simulink model "PMSM_MC_2025a"  (R2025a)
settings: Solver=FixedStepDiscrete  StartTime=0.0  StopTime=10.0  FixedStep=0.00005  RelTol=1e-3
values from neighbouring files (symbols this model uses):
  MC_DCurrLopKi_CFG = 0.008293758    [PMSM_MC_Data_2025a.sldd]
  MC_DCurrLopKp_CFG = 0.0870848    [PMSM_MC_Data_2025a.sldd]
  MC_MotModeDebug_CFG = 255.0    [PMSM_MC_Data_2025a.sldd]
  MC_POLE_NUM_CFG = 7.0    [PMSM_MC_Data_2025a.sldd]
  MC_QCurrLopKi_CFG = 0.008293758    [PMSM_MC_Data_2025a.sldd]
  MC_QCurrLopKp_CFG = 0.0870848    [PMSM_MC_Data_2025a.sldd]
  MC_SpdLopKi_CFG = 1.0E-5    [PMSM_MC_Data_2025a.sldd]
  MC_SpdLopKp_CFG = 0.002    [PMSM_MC_Data_2025a.sldd]
libraries: simulink x10, slpidlib x3
settings Model: DataDictionary=PMSM_MC_Data_2025a.sldd  Creator=EDY  LastModifiedBy=xiaoy
settings OptimizationCC: DefaultParameterBehavior=Inlined  EnhancedBackFolding=on  PassReuseOutputArgsAs=Individual arguments  ZeroExternalMemoryAtStartup=off  ZeroInternalMemoryAtStartup=off  OptimizeBlockOrder=speed  DifferentSizesBufferReuse=on  OptimizationCustomize=off  EfficientTunableParamExpr=on
settings DebuggingCC: ParameterTunabilityLossMsg=error
settings SFSimCC: MATLABDynamicMemAlloc=off
settings RTWCC: SystemTargetFile=ert.tlc  GenCodeOnly=on  TemplateMakefile=ert_default_tmf  GenerateReport=on  LaunchReport=on  Description=Embedded Coder
settings CodeAppCC: ForceParamTrailComments=on  IgnoreCustomStorageClasses=off  OperatorAnnotations=on  SimulinkDataObjDesc=on  SFDataObjDesc=on  InsertBlockDesc=on
settings ERTTargetCC: ExtModeTransport=0.0  ExtModeStaticAlloc=off  ExtModeMexFile=ext_comm  ExtModeIntrfLevel=Level1  ERTCustomFileTemplate=example_file_process.tlc  DynamicArrayContainerType=coder::array  TargetLangStandard=C99 (ISO)  GenerateSampleERTMain=on

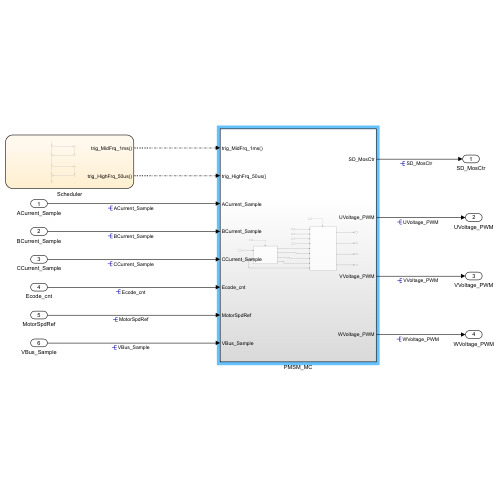
[thumbnail: Simulink's stored preview of the top-level diagram]
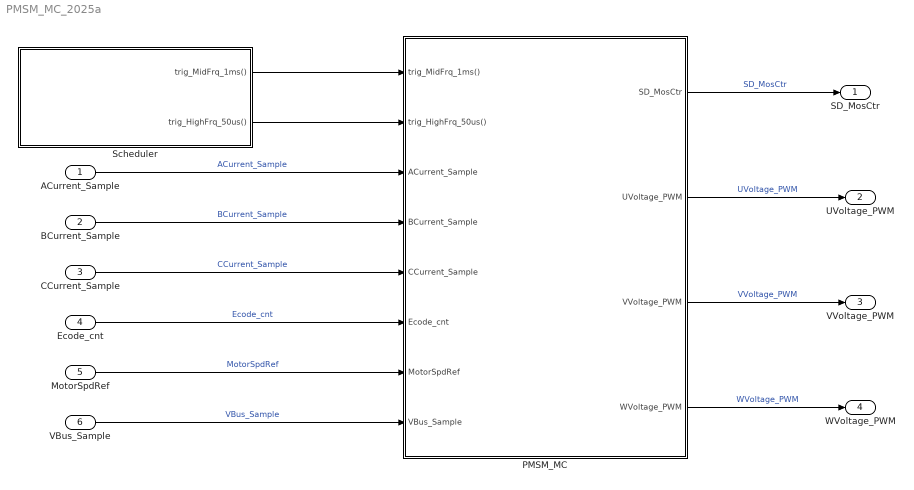
== system PMSM_MC_2025a ==
  ACurrent_Sample : Inport
  BCurrent_Sample : Inport  Port=2
  CCurrent_Sample : Inport  Port=3
  Ecode_cnt : Inport  Port=4
  MotorSpdRef : Inport  Port=5
  VBus_Sample : Inport  Port=6
  PMSM_MC : Subsystem
  Scheduler : Stateflow chart  TreatAsAtomicUnit=on
  SD_MosCtr : Outport
  UVoltage_PWM : Outport  Port=2
  VVoltage_PWM : Outport  Port=3
  WVoltage_PWM : Outport  Port=4
  wires:
  Scheduler/1(trig_MidFrq_1ms()) -> PMSM_MC/1(trig_MidFrq_1ms())
  Scheduler/2(trig_HighFrq_50us()) -> PMSM_MC/2(trig_HighFrq_50us())
  VBus_Sample/1 -> PMSM_MC/8(VBus_Sample)  "VBus_Sample"
  MotorSpdRef/1 -> PMSM_MC/7(MotorSpdRef)  "MotorSpdRef"
  Ecode_cnt/1 -> PMSM_MC/6(Ecode_cnt)  "Ecode_cnt"
  CCurrent_Sample/1 -> PMSM_MC/5(CCurrent_Sample)  "CCurrent_Sample"
  BCurrent_Sample/1 -> PMSM_MC/4(BCurrent_Sample)  "BCurrent_Sample"
  ACurrent_Sample/1 -> PMSM_MC/3(ACurrent_Sample)  "ACurrent_Sample"
  PMSM_MC/2(UVoltage_PWM) -> UVoltage_PWM/1  "UVoltage_PWM"
  PMSM_MC/1(SD_MosCtr) -> SD_MosCtr/1  "SD_MosCtr"
  PMSM_MC/3(VVoltage_PWM) -> VVoltage_PWM/1  "VVoltage_PWM"
  PMSM_MC/4(WVoltage_PWM) -> WVoltage_PWM/1  "WVoltage_PWM"

== system PMSM_MC_2025a/PMSM_MC ==
  trig_MidFrq_1ms() : Inport
  trig_HighFrq_50us() : Inport  Port=2
  ACurrent_Sample : Inport  Port=3
  BCurrent_Sample : Inport  Port=4
  CCurrent_Sample : Inport  Port=5
  Ecode_cnt : Inport  Port=6
  MotorSpdRef : Inport  Port=7
  VBus_Sample : Inport  Port=8
  MC_HighFrqTask : Subsystem  TreatAsAtomicUnit=on
  MC_LowFrqTask : Subsystem  TreatAsAtomicUnit=on
  SD_MosCtr : Outport
  UVoltage_PWM : Outport  Port=2
  VVoltage_PWM : Outport  Port=3
  WVoltage_PWM : Outport  Port=4
  wires:
  trig_MidFrq_1ms()/1 -> MC_LowFrqTask/Trigger
  trig_HighFrq_50us()/1 -> MC_HighFrqTask/Trigger
  Ecode_cnt/1 -> MC_HighFrqTask/9(Ecode_cnt), MC_LowFrqTask/2(Ecode_cnt)
  MotorSpdRef/1 -> MC_LowFrqTask/1(MotorSpdRef)
  ACurrent_Sample/1 -> MC_HighFrqTask/1(ACurrent_Sample)
  BCurrent_Sample/1 -> MC_HighFrqTask/2(BCurrent_Sample)
  CCurrent_Sample/1 -> MC_HighFrqTask/3(CCurrent_Sample)
  VBus_Sample/1 -> MC_HighFrqTask/4(VBus_Sample)
  MC_LowFrqTask/1(QAxiCurrent_Ref) -> MC_HighFrqTask/5(QAxiCurrent_Ref)
  MC_LowFrqTask/2(MotCalThetae) -> MC_HighFrqTask/6(MotCalThetae)
  MC_LowFrqTask/3(MotOffset) -> MC_HighFrqTask/7(MotOffset)
  MC_LowFrqTask/4(MotCtrMode) -> MC_HighFrqTask/8(MotCtrMode)
  MC_HighFrqTask/1(SD_MosCtr) -> SD_MosCtr/1
  MC_HighFrqTask/2(UVoltage_PWM) -> UVoltage_PWM/1
  MC_HighFrqTask/3(VVoltage_PWM) -> VVoltage_PWM/1
  MC_HighFrqTask/4(WVoltage_PWM) -> WVoltage_PWM/1

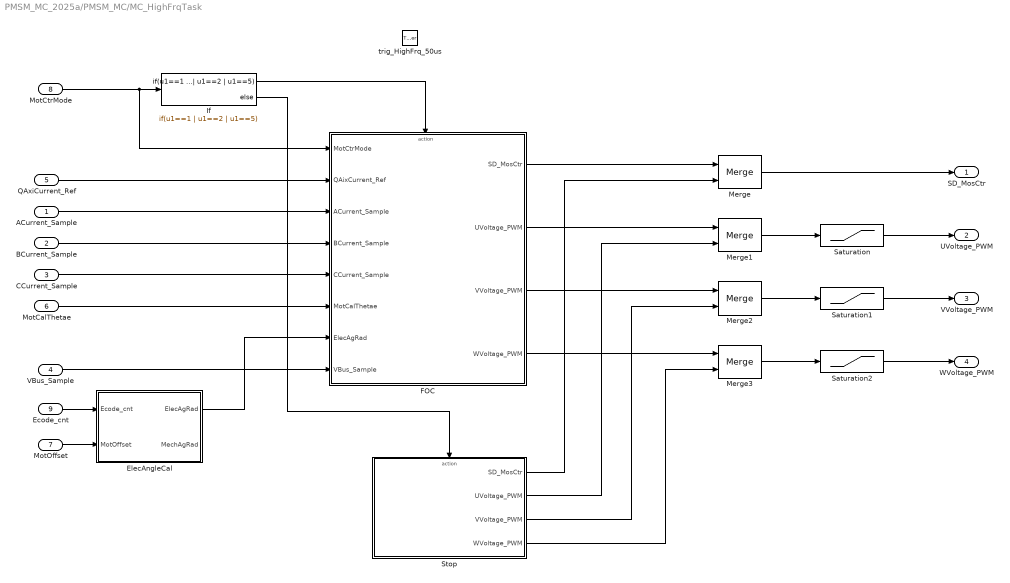
== system PMSM_MC_2025a/PMSM_MC/MC_HighFrqTask ==
  ACurrent_Sample : Inport
  BCurrent_Sample : Inport  Port=2
  CCurrent_Sample : Inport  Port=3
  VBus_Sample : Inport  Port=4
  QAxiCurrent_Ref : Inport  Port=5
  MotCalThetae : Inport  Port=6
  MotOffset : Inport  Port=7
  MotCtrMode : Inport  Port=8
  Ecode_cnt : Inport  Port=9
  trig_HighFrq_50us : TriggerPort  TriggerType=function-call  VariantControl=(inherit)
  ElecAngleCal : Subsystem
  FOC : Subsystem
  If : If  IfExpression=u1==1 | u1==2 | u1==5
  Merge{,1..3} (4 alike) : Merge
  Saturation : Saturate  UpperLimit=0.95  LowerLimit=0
      settings: AttributesFormatString=|
      | Upper = %<UpperLimit>
      | Lower = %<LowerLimit>
  Saturation1 : Saturate  UpperLimit=0.95  LowerLimit=0
      settings: AttributesFormatString=|
      | Upper = %<UpperLimit>
      | Lower = %<LowerLimit>
  Saturation2 : Saturate  UpperLimit=0.95  LowerLimit=0
      settings: AttributesFormatString=|
      | Upper = %<UpperLimit>
      | Lower = %<LowerLimit>
  Stop : Subsystem  TreatAsAtomicUnit=on
  SD_MosCtr : Outport
  UVoltage_PWM : Outport  Port=2
  VVoltage_PWM : Outport  Port=3
  WVoltage_PWM : Outport  Port=4
  wires:
  MotCtrMode/1 -> FOC/1(MotCtrMode), If/1
  If/1 -> FOC/Action
  If/2 -> Stop/Action
  FOC/1(SD_MosCtr) -> Merge/1
  FOC/2(UVoltage_PWM) -> Merge1/1
  FOC/3(VVoltage_PWM) -> Merge2/1
  FOC/4(WVoltage_PWM) -> Merge3/1
  Merge/1 -> SD_MosCtr/1
  Stop/1(SD_MosCtr) -> Merge/2
  Stop/2(UVoltage_PWM) -> Merge1/2
  Stop/3(VVoltage_PWM) -> Merge2/2
  Stop/4(WVoltage_PWM) -> Merge3/2
  Merge1/1 -> Saturation/1
  Merge3/1 -> Saturation2/1
  Merge2/1 -> Saturation1/1
  Saturation/1 -> UVoltage_PWM/1
  Saturation1/1 -> VVoltage_PWM/1
  Saturation2/1 -> WVoltage_PWM/1
  MotOffset/1 -> ElecAngleCal/2(MotOffset)
  Ecode_cnt/1 -> ElecAngleCal/1(Ecode_cnt)
  ACurrent_Sample/1 -> FOC/3(ACurrent_Sample)
  BCurrent_Sample/1 -> FOC/4(BCurrent_Sample)
  CCurrent_Sample/1 -> FOC/5(CCurrent_Sample)
  QAxiCurrent_Ref/1 -> FOC/2(QAixCurrent_Ref)
  MotCalThetae/1 -> FOC/6(MotCalThetae)
  VBus_Sample/1 -> FOC/8(VBus_Sample)
  ElecAngleCal/1(ElecAgRad) -> FOC/7(ElecAgRad)

== system PMSM_MC_2025a/PMSM_MC/MC_LowFrqTask ==
  MotorSpdRef : Inport
  Ecode_cnt : Inport  Port=2
  trig_MidFrq_1ms : TriggerPort  TriggerType=function-call  VariantControl=(inherit)
  MotModeCtr : Subsystem
  MotSpdCal : Subsystem
  SpdLoop : Subsystem
  QAxiCurrent_Ref : Outport
  MotCalThetae : Outport  Port=2
  MotOffset : Outport  Port=3
  MotCtrMode : Outport  Port=4
  wires:
  SpdLoop/1(QAxiCurrent_Ref) -> QAxiCurrent_Ref/1
  MotorSpdRef/1 -> SpdLoop/2(MotorSpdRef), MotModeCtr/2(MotorSpdRef)
  Ecode_cnt/1 -> MotSpdCal/1(Ecode_cnt), MotModeCtr/1(Ecode_cnt)
  MotSpdCal/1(MotorActSpd) -> SpdLoop/3(MotorActSpd)  "MotorActSpd"
  MotModeCtr/3(MotCtrMode) -> SpdLoop/1(MotCtrMode), MotCtrMode/1
  MotModeCtr/2(MotCalThetae) -> MotCalThetae/1
  MotModeCtr/1(MotOffset) -> MotOffset/1

== system PMSM_MC_2025a/PMSM_MC/MC_HighFrqTask/ElecAngleCal ==
  Ecode_cnt : Inport
  MotOffset : Inport  Port=2
  Add : Sum  Inputs=+-
  AngleCal : Subsystem
  Demux : Demux  Outputs=2
  ElecAgRad : Outport
  MechAgRad : Outport  Port=2
  wires:
  Ecode_cnt/1 -> Add/1
  MotOffset/1 -> Add/2
  Add/1 -> AngleCal/1(Ecode_CntCorrect)
  AngleCal/1(Theta) -> Demux/1
  Demux/1 -> MechAgRad/1
  Demux/2 -> ElecAgRad/1

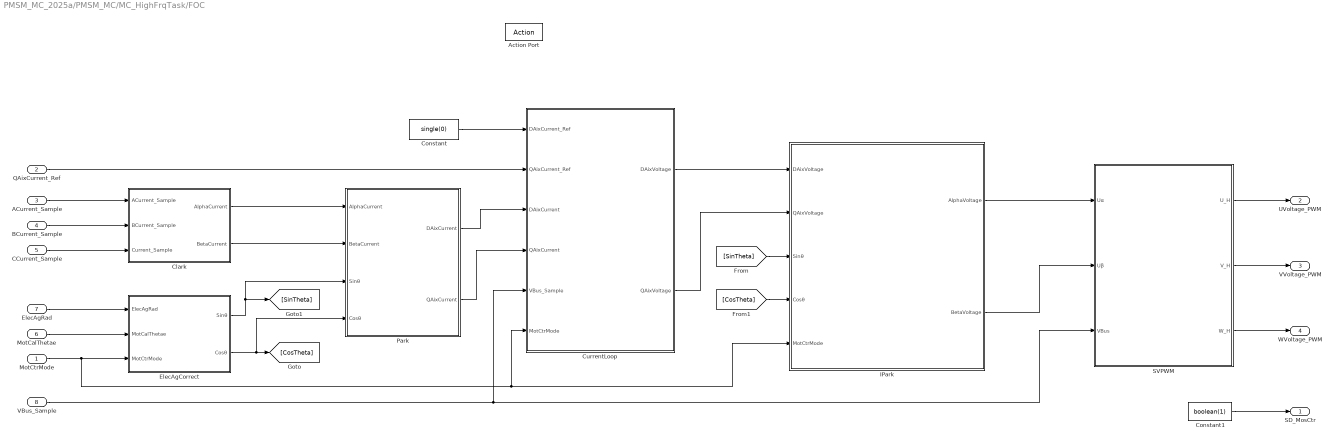
== system PMSM_MC_2025a/PMSM_MC/MC_HighFrqTask/FOC ==
  MotCtrMode : Inport
  QAixCurrent_Ref : Inport  Port=2
  ACurrent_Sample : Inport  Port=3
  BCurrent_Sample : Inport  Port=4
  CCurrent_Sample : Inport  Port=5
  MotCalThetae : Inport  Port=6
  ElecAgRad : Inport  Port=7
  VBus_Sample : Inport  Port=8
  Action Port : ActionPort  ActionPortLabel=if(u1==1 | u1==2 | u1==5)
  Clark : Subsystem
  Constant : Constant  Value=single(0)
  Constant1 : Constant  Value=boolean(1)
  CurrentLoop : Subsystem
  ElecAgCorrect : Subsystem
  IPark : Subsystem
  Park : Subsystem
  SVPWM : Subsystem
  SD_MosCtr : Outport
  UVoltage_PWM : Outport  Port=2
  VVoltage_PWM : Outport  Port=3
  WVoltage_PWM : Outport  Port=4
  wires:
  Clark/2(BetaCurrent) -> Park/2(BetaCurrent)
  Clark/1(AlphaCurrent) -> Park/1(AlphaCurrent)
  Park/1(DAixCurrent) -> CurrentLoop/3(DAixCurrent)
  QAixCurrent_Ref/1 -> CurrentLoop/2(QAixCurrent_Ref)
  Constant/1 -> CurrentLoop/1(DAixCurrent_Ref)
  CurrentLoop/1(DAixVoltage) -> IPark/1(DAixVoltage)
  CurrentLoop/2(QAixVoltage) -> IPark/2(QAixVoltage)
  Park/2(QAixCurrent) -> CurrentLoop/4(QAixCurrent)
  ACurrent_Sample/1 -> Clark/1(ACurrent_Sample)
  BCurrent_Sample/1 -> Clark/2(BCurrent_Sample)
  CCurrent_Sample/1 -> Clark/3(Current_Sample)
  ElecAgRad/1 -> ElecAgCorrect/1(ElecAgRad)
  MotCalThetae/1 -> ElecAgCorrect/2(MotCalThetae)
  MotCtrMode/1 -> CurrentLoop/6(MotCtrMode), IPark/5(MotCtrMode), ElecAgCorrect/3(MotCtrMode)
  ElecAgCorrect/1(Sinθ) -> Park/3(Sinθ), [SinTheta]
  ElecAgCorrect/2(Cosθ) -> [CosTheta], Park/4(Cosθ)
  [SinTheta] -> IPark/3(Sinθ)
  [CosTheta] -> IPark/4(Cosθ)
  VBus_Sample/1 -> CurrentLoop/5(VBus_Sample), SVPWM/3(VBus)
  IPark/1(AlphaVoltage) -> SVPWM/1(Uα)
  IPark/2(BetaVoltage) -> SVPWM/2(Uβ)
  SVPWM/1(U_H) -> UVoltage_PWM/1
  SVPWM/2(V_H) -> VVoltage_PWM/1
  SVPWM/3(W_H) -> WVoltage_PWM/1
  Constant1/1 -> SD_MosCtr/1

== system PMSM_MC_2025a/PMSM_MC/MC_HighFrqTask/Stop ==
  Action Port : ActionPort  ActionPortLabel=else
  Constant : Constant  Value=single(0)
  Constant1 : Constant  Value=boolean(0)
  SD_MosCtr : Outport
  UVoltage_PWM : Outport  Port=2
  VVoltage_PWM : Outport  Port=3
  WVoltage_PWM : Outport  Port=4
  wires:
  Constant/1 -> WVoltage_PWM/1, VVoltage_PWM/1, UVoltage_PWM/1
  Constant1/1 -> SD_MosCtr/1

== system PMSM_MC_2025a/PMSM_MC/MC_LowFrqTask/MotModeCtr ==
  Ecode_cnt : Inport
  MotorSpdRef : Inport  Port=2
  Chart : Stateflow chart  TreatAsAtomicUnit=on
  Compare To Constant : simulink/Logic and Bit Operations/Compare To Constant  relop=~=  const=255  OutDataTypeStr=boolean
  Constant : Constant  Value=MC_MotModeDebug_CFG
  Switch : Switch  Criteria=u2 ~= 0  SaturateOnIntegerOverflow=off  InputSameDT=off
  MotOffset : Outport
  MotCalThetae : Outport  Port=2
  MotCtrMode : Outport  Port=3
  wires:
  Chart/2(MotOffset) -> MotOffset/1
  Chart/3(MotCalThetae) -> MotCalThetae/1
  Ecode_cnt/1 -> Chart/1(Ecode_cnt)
  MotorSpdRef/1 -> Chart/2(MotorSpdRef)
  Chart/1(MotCtrMode) -> Switch/3
  Switch/1 -> MotCtrMode/1
  Constant/1 -> Switch/1, Compare To Constant/1
  Compare To Constant/1 -> Switch/2

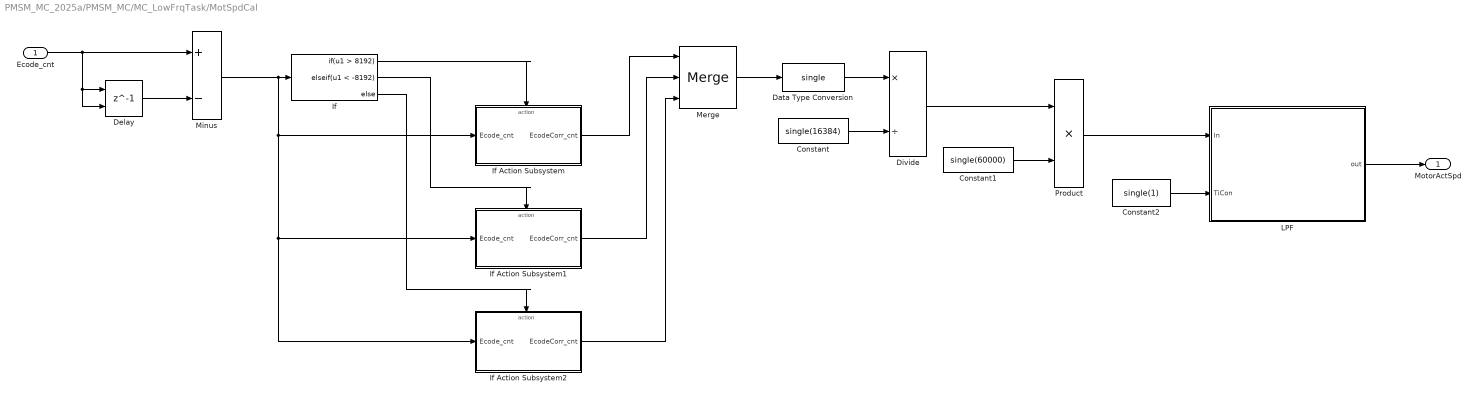
== system PMSM_MC_2025a/PMSM_MC/MC_LowFrqTask/MotSpdCal ==
  Ecode_cnt : Inport
  Constant : Constant  Value=single(16384)
  Constant1 : Constant  Value=single(60000)
  Constant2 : Constant  Value=single(1)
  Data Type Conversion : DataTypeConversion  OutDataTypeStr=single  SaturateOnIntegerOverflow=off  RndMeth=Floor
  Delay : Delay  DelayLength=1  InitialConditionSource=Input port
      settings: InputPortMap=u0,p4
  Divide : Product  Inputs=*/
  If : If  IfExpression=u1 > 8192  ElseIfExpressions=u1 < -8192
  If Action Subsystem : Subsystem  TreatAsAtomicUnit=on
  If Action Subsystem1 : Subsystem  TreatAsAtomicUnit=on
  If Action Subsystem2 : Subsystem  TreatAsAtomicUnit=on
  LPF : Subsystem
  Merge : Merge  Inputs=3
  Minus : Sum  Inputs=+-
  Product : Product
  MotorActSpd : Outport
  wires:
  Ecode_cnt/1 -> Delay/2, Delay/1, Minus/1
  Delay/1 -> Minus/2
  Data Type Conversion/1 -> Divide/1
  Constant/1 -> Divide/2
  Divide/1 -> Product/1
  Constant1/1 -> Product/2
  Product/1 -> LPF/1(In)
  Constant2/1 -> LPF/2(TiCon)
  LPF/1(out) -> MotorActSpd/1
  Minus/1 -> If Action Subsystem/1(Ecode_cnt), If Action Subsystem2/1(Ecode_cnt), If Action Subsystem1/1(Ecode_cnt), If/1
  If/1 -> If Action Subsystem/Action
  If/2 -> If Action Subsystem1/Action
  If/3 -> If Action Subsystem2/Action
  If Action Subsystem/1(EcodeCorr_cnt) -> Merge/1
  If Action Subsystem1/1(EcodeCorr_cnt) -> Merge/2
  If Action Subsystem2/1(EcodeCorr_cnt) -> Merge/3
  Merge/1 -> Data Type Conversion/1

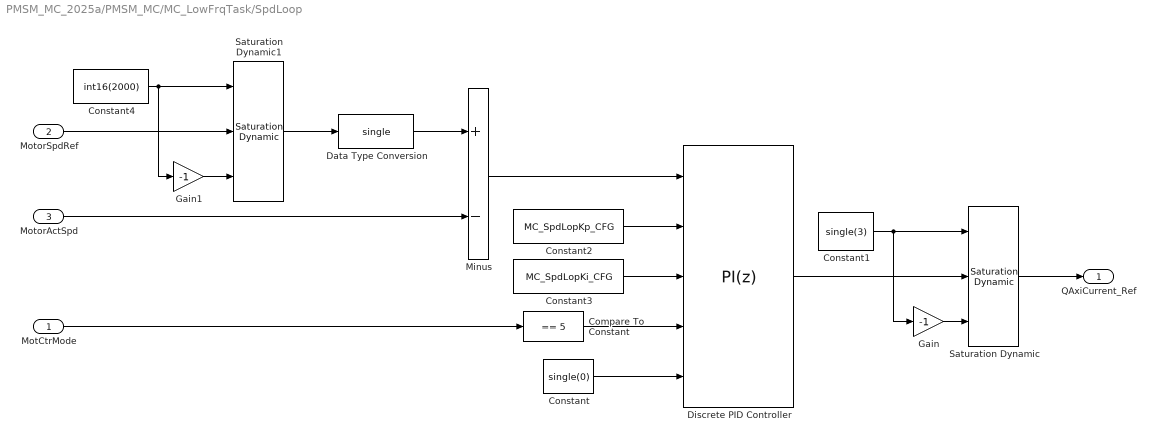
== system PMSM_MC_2025a/PMSM_MC/MC_LowFrqTask/SpdLoop ==
  MotCtrMode : Inport
  MotorSpdRef : Inport  Port=2
  MotorActSpd : Inport  Port=3
  Compare To Constant : simulink/Logic and Bit Operations/Compare To Constant  relop===  const=5  OutDataTypeStr=boolean
  Constant : Constant  Value=single(0)  OutDataTypeStr=single
  Constant1 : Constant  Value=single(3)
  Constant2 : Constant  Value=MC_SpdLopKp_CFG
  Constant3 : Constant  Value=MC_SpdLopKi_CFG
  Constant4 : Constant  Value=int16(2000)
  Data Type Conversion : DataTypeConversion  OutDataTypeStr=single  SaturateOnIntegerOverflow=off  RndMeth=Floor
  Discrete PID Controller : slpidlib/PID Controller  Controller=PI  Form=Parallel  TimeDomain=Discrete-time  UseExternalTs=off  SampleTime=-1  IntegratorMethod=Forward Euler  FilterMethod=Forward Euler  ControllerParametersSource=external  P=1  I=1  UseKiTs=on  D=0  UseExternalDerivativeSource=off  N=100  UseFilter=on  TunerSelectOption=Transfer Function Based (PID Tuner App)  InitialConditionSource=external  InitialConditionForIntegrator=0  InitialConditionForFilter=0  DifferentiatorICPrevScaledInput=0  ExternalReset=rising  TrackingMode=off  Kt=1  LimitOutput=off  SatLimitsSource=external  UpperSaturationLimit=inf  LowerSaturationLimit=-inf  LinearizeAsGain=off  AntiWindupMode=none  Kb=1  LimitIntegrator=on  UpperIntegratorSaturationLimit=3  LowerIntegratorSaturationLimit=-3  POutMin=[]  POutMax=[]  IOutMin=[]  IOutMax=[]  DOutMin=[]  DOutMax=[]  NOutMin=[]  NOutMax=[]  SumOutMin=[]  SumOutMax=[]  SaturationOutMin=[]  SaturationOutMax=[]  PParamMin=[]  PParamMax=[]  IParamMin=[]  IParamMax=[]  DParamMin=[]  DParamMax=[]  NParamMin=[]  NParamMax=[]  KbParamMin=[]  KbParamMax=[]  KtParamMin=[]  KtParamMax=[]  KbOutMin=[]  KbOutMax=[]  KtOutMin=[]  KtOutMax=[]  IntegratorOutMin=[]  IntegratorOutMax=[]  FilterOutMin=[]  FilterOutMax=[]  SumI1OutMin=[]  SumI1OutMax=[]  SumI2OutMin=[]  SumI2OutMax=[]  SumI3OutMin=[]  SumI3OutMax=[]  SumI4OutMin=[]  SumI4OutMax=[]  SumDOutMin=[]  SumDOutMax=[]  DifferentiatorOutMin=[]  DifferentiatorOutMax=[]  FilterDiffOutCoefMin=[]  FilterDiffOutCoefMax=[]  ReciprocalOutMin=[]  ReciprocalOutMax=[]  SumDenOutMin=[]  SumDenOutMax=[]  SumNumOutMin=[]  SumNumOutMax=[]  DivideOutMin=[]  DivideOutMax=[]  UdiffTsProdOutMin=[]  UdiffTsProdOutMax=[]  NTsProdOutMin=[]  NTsProdOutMax=[]  UintegralTsProdOutMin=[]  UintegralTsProdOutMax=[]  UngainTsProdOutMin=[]  UngainTsProdOutMax=[]  ClampingZeroOutDataTypeStr=Inherit: Inherit via back propagation  ClampingZeroOutMin=[]  ClampingZeroOutMax=[]  FilterDenConstantOutDataTypeStr=Inherit: Inherit via back propagation  FilterDenConstantOutMin=[]  FilterDenConstantOutMax=[]  PCopyOutDataTypeStr=Inherit: Inherit via back propagation  PCopyOutMin=[]  PCopyOutMax=[]  NCopyOutDataTypeStr=Inherit: Inherit via back propagation  NCopyOutMin=[]  NCopyOutMax=[]  IntegratorContinuousStateAttributes=''  IntegratorStateMustResolveToSignalObject=off  IntegratorRTWStateStorageClass=Auto  FilterContinuousStateAttributes=''  FilterStateMustResolveToSignalObject=off  FilterRTWStateStorageClass=Auto  ParallelPVariant=ExternalParameters  IdealPVariant=Disabled  IVariant=ExternalParameters  DVariant=Disabled  IntegratorVariant=Discrete  SatVariant=Disabled  AWVariant=Passthrough  PCopyVariant=Disabled  TRVariant=Disabled  FdbkBlocksVariant=Forward  IdealPFdbkVariant=Disabled  SatFdbkVariant=Disabled  DerivativeFilterVariant=Disabled  NVariant=Disabled  NCopyVariant=Disabled_SignalSpec  FilterICVariant=Disabled  IntegratorICVariant=ExternalICs  ExternalResetVariant=ExternalReset  TRSumVariant=Passthrough  SumFdbkVariant=Disabled  SumVariant=Sum_PI  TsampFilterVariant=InternalTs  TsampNgainVariant=Passthrough  TsampIntegralVariant=Disabled_SignalSpec  ExternalSaturationOutDataTypeStr=Inherit: Same as second input  DerivativeSourceVariant=Disabled  PreIntVariant=InternalPreInt
      settings: LibrarySourceBlock=simulink/Discrete/Discrete PID Controller
  Gain : Gain  Gain=-1
  Gain1 : Gain  Gain=-1
  Minus : Sum  Inputs=+-
  Saturation Dynamic : simulink/Discontinuities/Saturation Dynamic  OutMin=[]  OutMax=[]  OutDataTypeStr=Inherit: Same as second input  OutDataType=fixdt(1, 16)  OutScaling=2^-10  DoSatur=off
  Saturation Dynamic1 : simulink/Discontinuities/Saturation Dynamic  OutMin=[]  OutMax=[]  OutDataTypeStr=Inherit: Same as second input  OutDataType=fixdt(1, 16)  OutScaling=2^-10  DoSatur=off
  QAxiCurrent_Ref : Outport
  wires:
  Data Type Conversion/1 -> Minus/1
  Constant/1 -> Discrete PID Controller/5
  Discrete PID Controller/1 -> Saturation Dynamic/2
  Saturation Dynamic/1 -> QAxiCurrent_Ref/1
  Constant1/1 -> Saturation Dynamic/1, Gain/1
  Gain/1 -> Saturation Dynamic/3
  Minus/1 -> Discrete PID Controller/1
  Constant2/1 -> Discrete PID Controller/2
  Constant3/1 -> Discrete PID Controller/3
  MotorSpdRef/1 -> Saturation Dynamic1/2
  Saturation Dynamic1/1 -> Data Type Conversion/1
  Constant4/1 -> Gain1/1, Saturation Dynamic1/1
  Gain1/1 -> Saturation Dynamic1/3
  MotorActSpd/1 -> Minus/2
  Compare To Constant/1 -> Discrete PID Controller/4
  MotCtrMode/1 -> Compare To Constant/1

== system PMSM_MC_2025a/PMSM_MC/MC_HighFrqTask/ElecAngleCal/AngleCal ==
  Ecode_CntCorrect : Inport
  If : If  IfExpression=u1 == 1  ElseIfExpressions=u1 == -1
  If Action Subsystem : Subsystem  TreatAsAtomicUnit=on
  If Action Subsystem1 : Subsystem  TreatAsAtomicUnit=on
  If Action Subsystem2 : Subsystem  TreatAsAtomicUnit=on
  Merge : Merge  Inputs=3
  Sign : Signum
  Theta : Outport
  wires:
  Ecode_CntCorrect/1 -> If Action Subsystem1/1(Ecode_PhyVal), If Action Subsystem/1(Ecode_PhyVal), Sign/1
  Sign/1 -> If/1
  If/1 -> If Action Subsystem/Action
  If/2 -> If Action Subsystem1/Action
  If/3 -> If Action Subsystem2/Action
  If Action Subsystem1/1(Out1) -> Merge/2
  If Action Subsystem/1(Out1) -> Merge/1
  Merge/1 -> Theta/1
  If Action Subsystem2/1(Out1) -> Merge/3

== system PMSM_MC_2025a/PMSM_MC/MC_HighFrqTask/FOC/Clark ==
  ACurrent_Sample : Inport
  BCurrent_Sample : Inport  Port=2
  Current_Sample : Inport  Port=3
  Gain : Gain  Gain=0.57735
  Gain1 : Gain  Gain=0.57735
  Minus : Sum  Inputs=+-
  AlphaCurrent : Outport
  BetaCurrent : Outport  Port=2
  wires:
  ACurrent_Sample/1 -> AlphaCurrent/1
  Minus/1 -> BetaCurrent/1
  Gain1/1 -> Minus/2
  Gain/1 -> Minus/1
  BCurrent_Sample/1 -> Gain/1
  Current_Sample/1 -> Gain1/1

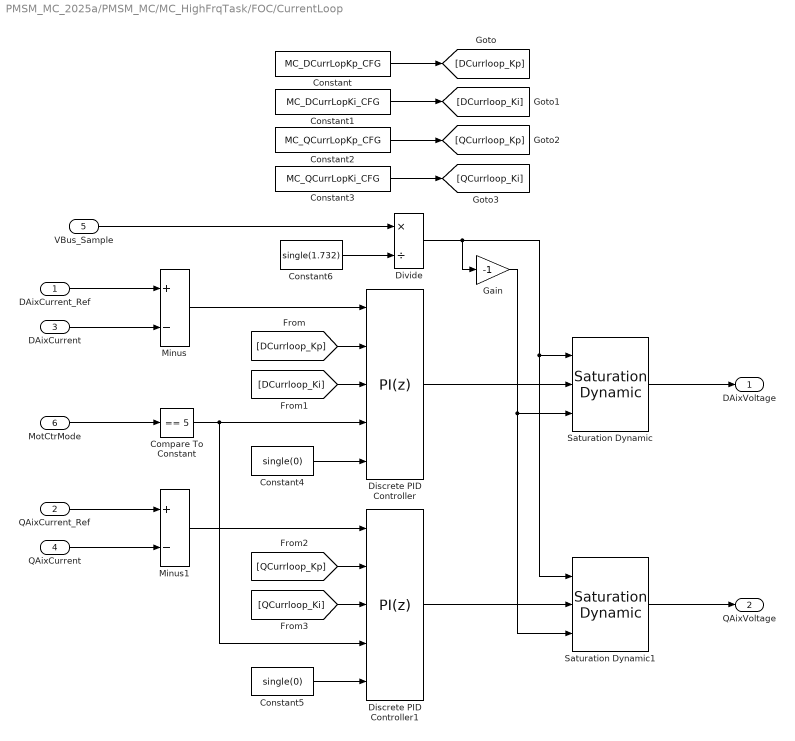
== system PMSM_MC_2025a/PMSM_MC/MC_HighFrqTask/FOC/CurrentLoop ==
  DAixCurrent_Ref : Inport
  QAixCurrent_Ref : Inport  Port=2
  DAixCurrent : Inport  Port=3
  QAixCurrent : Inport  Port=4
  VBus_Sample : Inport  Port=5
  MotCtrMode : Inport  Port=6
  Compare To Constant : simulink/Logic and Bit Operations/Compare To Constant  relop===  const=5  OutDataTypeStr=boolean
  Constant : Constant  Value=MC_DCurrLopKp_CFG
  Constant1 : Constant  Value=MC_DCurrLopKi_CFG
  Constant2 : Constant  Value=MC_QCurrLopKp_CFG
  Constant3 : Constant  Value=MC_QCurrLopKi_CFG
  Constant4 : Constant  Value=single(0)
  Constant5 : Constant  Value=single(0)
  Constant6 : Constant  Value=single(1.732)
  Discrete PID Controller : slpidlib/PID Controller  Controller=PI  Form=Parallel  TimeDomain=Discrete-time  UseExternalTs=off  SampleTime=-1  IntegratorMethod=Forward Euler  FilterMethod=Forward Euler  ControllerParametersSource=external  P=1  I=1  UseKiTs=on  D=0  UseExternalDerivativeSource=off  N=100  UseFilter=on  TunerSelectOption=Transfer Function Based (PID Tuner App)  InitialConditionSource=external  InitialConditionForIntegrator=0  InitialConditionForFilter=0  DifferentiatorICPrevScaledInput=0  ExternalReset=rising  TrackingMode=off  Kt=1  LimitOutput=off  SatLimitsSource=internal  UpperSaturationLimit=inf  LowerSaturationLimit=-inf  LinearizeAsGain=off  AntiWindupMode=none  Kb=1  LimitIntegrator=on  UpperIntegratorSaturationLimit=13  LowerIntegratorSaturationLimit=-13  POutMin=[]  POutMax=[]  IOutMin=[]  IOutMax=[]  DOutMin=[]  DOutMax=[]  NOutMin=[]  NOutMax=[]  SumOutMin=[]  SumOutMax=[]  SaturationOutMin=[]  SaturationOutMax=[]  PParamMin=[]  PParamMax=[]  IParamMin=[]  IParamMax=[]  DParamMin=[]  DParamMax=[]  NParamMin=[]  NParamMax=[]  KbParamMin=[]  KbParamMax=[]  KtParamMin=[]  KtParamMax=[]  KbOutMin=[]  KbOutMax=[]  KtOutMin=[]  KtOutMax=[]  IntegratorOutMin=[]  IntegratorOutMax=[]  FilterOutMin=[]  FilterOutMax=[]  SumI1OutMin=[]  SumI1OutMax=[]  SumI2OutMin=[]  SumI2OutMax=[]  SumI3OutMin=[]  SumI3OutMax=[]  SumI4OutMin=[]  SumI4OutMax=[]  SumDOutMin=[]  SumDOutMax=[]  DifferentiatorOutMin=[]  DifferentiatorOutMax=[]  FilterDiffOutCoefMin=[]  FilterDiffOutCoefMax=[]  ReciprocalOutMin=[]  ReciprocalOutMax=[]  SumDenOutMin=[]  SumDenOutMax=[]  SumNumOutMin=[]  SumNumOutMax=[]  DivideOutMin=[]  DivideOutMax=[]  UdiffTsProdOutMin=[]  UdiffTsProdOutMax=[]  NTsProdOutMin=[]  NTsProdOutMax=[]  UintegralTsProdOutMin=[]  UintegralTsProdOutMax=[]  UngainTsProdOutMin=[]  UngainTsProdOutMax=[]  ClampingZeroOutDataTypeStr=Inherit: Inherit via back propagation  ClampingZeroOutMin=[]  ClampingZeroOutMax=[]  FilterDenConstantOutDataTypeStr=Inherit: Inherit via back propagation  FilterDenConstantOutMin=[]  FilterDenConstantOutMax=[]  PCopyOutDataTypeStr=Inherit: Inherit via back propagation  PCopyOutMin=[]  PCopyOutMax=[]  NCopyOutDataTypeStr=Inherit: Inherit via back propagation  NCopyOutMin=[]  NCopyOutMax=[]  IntegratorContinuousStateAttributes=''  IntegratorStateMustResolveToSignalObject=off  IntegratorRTWStateStorageClass=Auto  FilterContinuousStateAttributes=''  FilterStateMustResolveToSignalObject=off  FilterRTWStateStorageClass=Auto  ParallelPVariant=ExternalParameters  IdealPVariant=Disabled  IVariant=ExternalParameters  DVariant=Disabled  IntegratorVariant=Discrete  SatVariant=Disabled  AWVariant=Passthrough  PCopyVariant=Disabled  TRVariant=Disabled  FdbkBlocksVariant=Forward  IdealPFdbkVariant=Disabled  SatFdbkVariant=Disabled  DerivativeFilterVariant=Disabled  NVariant=Disabled  NCopyVariant=Disabled_SignalSpec  FilterICVariant=Disabled  IntegratorICVariant=ExternalICs  ExternalResetVariant=ExternalReset  TRSumVariant=Passthrough  SumFdbkVariant=Disabled  SumVariant=Sum_PI  TsampFilterVariant=InternalTs  TsampNgainVariant=Passthrough  TsampIntegralVariant=Disabled_SignalSpec  ExternalSaturationOutDataTypeStr=Inherit: Same as second input  DerivativeSourceVariant=Disabled  PreIntVariant=InternalPreInt
      settings: LibrarySourceBlock=simulink/Discrete/Discrete PID Controller
  Discrete PID Controller1 : slpidlib/PID Controller  Controller=PI  Form=Parallel  TimeDomain=Discrete-time  UseExternalTs=off  SampleTime=-1  IntegratorMethod=Forward Euler  FilterMethod=Forward Euler  ControllerParametersSource=external  P=1  I=1  UseKiTs=on  D=0  UseExternalDerivativeSource=off  N=100  UseFilter=on  TunerSelectOption=Transfer Function Based (PID Tuner App)  InitialConditionSource=external  InitialConditionForIntegrator=0  InitialConditionForFilter=0  DifferentiatorICPrevScaledInput=0  ExternalReset=rising  TrackingMode=off  Kt=1  LimitOutput=off  SatLimitsSource=internal  UpperSaturationLimit=inf  LowerSaturationLimit=-inf  LinearizeAsGain=off  AntiWindupMode=none  Kb=1  LimitIntegrator=on  UpperIntegratorSaturationLimit=13  LowerIntegratorSaturationLimit=-13  POutMin=[]  POutMax=[]  IOutMin=[]  IOutMax=[]  DOutMin=[]  DOutMax=[]  NOutMin=[]  NOutMax=[]  SumOutMin=[]  SumOutMax=[]  SaturationOutMin=[]  SaturationOutMax=[]  PParamMin=[]  PParamMax=[]  IParamMin=[]  IParamMax=[]  DParamMin=[]  DParamMax=[]  NParamMin=[]  NParamMax=[]  KbParamMin=[]  KbParamMax=[]  KtParamMin=[]  KtParamMax=[]  KbOutMin=[]  KbOutMax=[]  KtOutMin=[]  KtOutMax=[]  IntegratorOutMin=[]  IntegratorOutMax=[]  FilterOutMin=[]  FilterOutMax=[]  SumI1OutMin=[]  SumI1OutMax=[]  SumI2OutMin=[]  SumI2OutMax=[]  SumI3OutMin=[]  SumI3OutMax=[]  SumI4OutMin=[]  SumI4OutMax=[]  SumDOutMin=[]  SumDOutMax=[]  DifferentiatorOutMin=[]  DifferentiatorOutMax=[]  FilterDiffOutCoefMin=[]  FilterDiffOutCoefMax=[]  ReciprocalOutMin=[]  ReciprocalOutMax=[]  SumDenOutMin=[]  SumDenOutMax=[]  SumNumOutMin=[]  SumNumOutMax=[]  DivideOutMin=[]  DivideOutMax=[]  UdiffTsProdOutMin=[]  UdiffTsProdOutMax=[]  NTsProdOutMin=[]  NTsProdOutMax=[]  UintegralTsProdOutMin=[]  UintegralTsProdOutMax=[]  UngainTsProdOutMin=[]  UngainTsProdOutMax=[]  ClampingZeroOutDataTypeStr=Inherit: Inherit via back propagation  ClampingZeroOutMin=[]  ClampingZeroOutMax=[]  FilterDenConstantOutDataTypeStr=Inherit: Inherit via back propagation  FilterDenConstantOutMin=[]  FilterDenConstantOutMax=[]  PCopyOutDataTypeStr=Inherit: Inherit via back propagation  PCopyOutMin=[]  PCopyOutMax=[]  NCopyOutDataTypeStr=Inherit: Inherit via back propagation  NCopyOutMin=[]  NCopyOutMax=[]  IntegratorContinuousStateAttributes=''  IntegratorStateMustResolveToSignalObject=off  IntegratorRTWStateStorageClass=Auto  FilterContinuousStateAttributes=''  FilterStateMustResolveToSignalObject=off  FilterRTWStateStorageClass=Auto  ParallelPVariant=ExternalParameters  IdealPVariant=Disabled  IVariant=ExternalParameters  DVariant=Disabled  IntegratorVariant=Discrete  SatVariant=Disabled  AWVariant=Passthrough  PCopyVariant=Disabled  TRVariant=Disabled  FdbkBlocksVariant=Forward  IdealPFdbkVariant=Disabled  SatFdbkVariant=Disabled  DerivativeFilterVariant=Disabled  NVariant=Disabled  NCopyVariant=Disabled_SignalSpec  FilterICVariant=Disabled  IntegratorICVariant=ExternalICs  ExternalResetVariant=ExternalReset  TRSumVariant=Passthrough  SumFdbkVariant=Disabled  SumVariant=Sum_PI  TsampFilterVariant=InternalTs  TsampNgainVariant=Passthrough  TsampIntegralVariant=Disabled_SignalSpec  ExternalSaturationOutDataTypeStr=Inherit: Same as second input  DerivativeSourceVariant=Disabled  PreIntVariant=InternalPreInt
      settings: LibrarySourceBlock=simulink/Discrete/Discrete PID Controller
  Divide : Product  Inputs=*/
  Gain : Gain  Gain=-1
  Minus : Sum  Inputs=+-
  Minus1 : Sum  Inputs=+-
  Saturation Dynamic : simulink/Discontinuities/Saturation Dynamic  OutMin=[]  OutMax=[]  OutDataTypeStr=Inherit: Same as second input  OutDataType=fixdt(1, 16)  OutScaling=2^-10  DoSatur=off
  Saturation Dynamic1 : simulink/Discontinuities/Saturation Dynamic  OutMin=[]  OutMax=[]  OutDataTypeStr=Inherit: Same as second input  OutDataType=fixdt(1, 16)  OutScaling=2^-10  DoSatur=off
  DAixVoltage : Outport
  QAixVoltage : Outport  Port=2
  wires:
  Minus/1 -> Discrete PID Controller/1
  DAixCurrent_Ref/1 -> Minus/1
  DAixCurrent/1 -> Minus/2
  QAixCurrent/1 -> Minus1/2
  QAixCurrent_Ref/1 -> Minus1/1
  Minus1/1 -> Discrete PID Controller1/1
  Constant/1 -> [DCurrloop_Kp]
  Constant1/1 -> [DCurrloop_Ki]
  Constant2/1 -> [QCurrloop_Kp]
  Constant3/1 -> [QCurrloop_Ki]
  [DCurrloop_Kp] -> Discrete PID Controller/2
  [DCurrloop_Ki] -> Discrete PID Controller/3
  Constant4/1 -> Discrete PID Controller/5
  [QCurrloop_Kp] -> Discrete PID Controller1/2
  [QCurrloop_Ki] -> Discrete PID Controller1/3
  Constant5/1 -> Discrete PID Controller1/5
  Constant6/1 -> Divide/2
  VBus_Sample/1 -> Divide/1
  Divide/1 -> Gain/1, Saturation Dynamic1/1, Saturation Dynamic/1
  Discrete PID Controller/1 -> Saturation Dynamic/2
  Discrete PID Controller1/1 -> Saturation Dynamic1/2
  Saturation Dynamic/1 -> DAixVoltage/1
  Saturation Dynamic1/1 -> QAixVoltage/1
  Gain/1 -> Saturation Dynamic1/3, Saturation Dynamic/3
  MotCtrMode/1 -> Compare To Constant/1
  Compare To Constant/1 -> Discrete PID Controller1/4, Discrete PID Controller/4

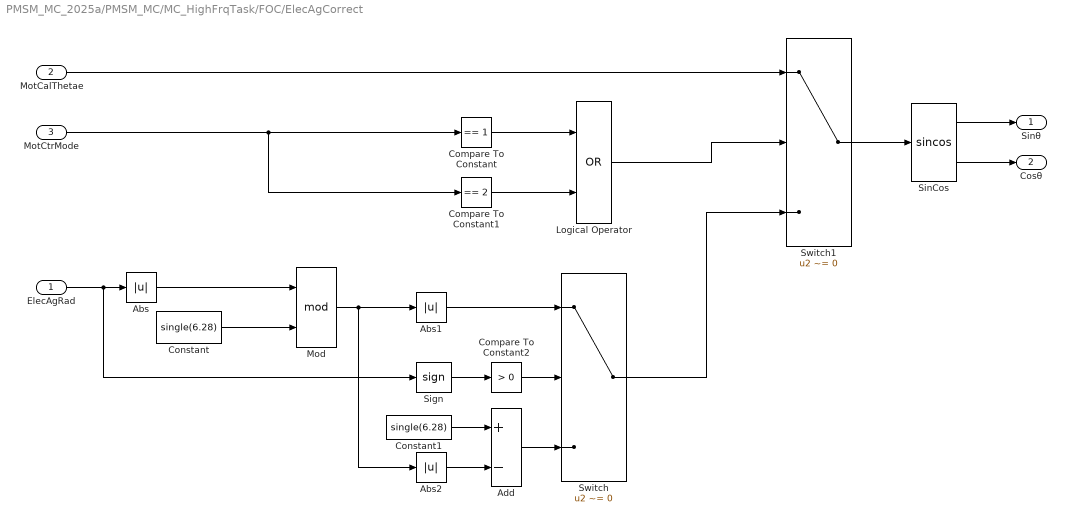
== system PMSM_MC_2025a/PMSM_MC/MC_HighFrqTask/FOC/ElecAgCorrect ==
  ElecAgRad : Inport
  MotCalThetae : Inport  Port=2
  MotCtrMode : Inport  Port=3
  Abs : Abs  SaturateOnIntegerOverflow=off
  Abs1 : Abs  SaturateOnIntegerOverflow=off
  Abs2 : Abs  SaturateOnIntegerOverflow=off
  Add : Sum  Inputs=+-
  Compare To Constant : simulink/Logic and Bit Operations/Compare To Constant  relop===  const=1  OutDataTypeStr=boolean
  Compare To Constant1 : simulink/Logic and Bit Operations/Compare To Constant  relop===  const=2  OutDataTypeStr=boolean
  Compare To Constant2 : simulink/Logic and Bit Operations/Compare To Constant  relop=>  const=0  OutDataTypeStr=boolean
  Constant : Constant  Value=single(6.28)
  Constant1 : Constant  Value=single(6.28)
  Logical Operator : Logic  Operator=OR  AllPortsSameDT=off  OutDataTypeStr=boolean
  Mod : Math  Operator=mod
  Sign : Signum
  SinCos : Trigonometry  Operator=sincos
  Switch : Switch  Criteria=u2 ~= 0  SaturateOnIntegerOverflow=off  InputSameDT=off
  Switch1 : Switch  Criteria=u2 ~= 0  SaturateOnIntegerOverflow=off  InputSameDT=off
  Sinθ : Outport
  Cosθ : Outport  Port=2
  wires:
  ElecAgRad/1 -> Abs/1, Sign/1
  Constant/1 -> Mod/2
  Abs/1 -> Mod/1
  Mod/1 -> Abs2/1, Abs1/1
  MotCtrMode/1 -> Compare To Constant1/1, Compare To Constant/1
  Compare To Constant/1 -> Logical Operator/1
  Compare To Constant1/1 -> Logical Operator/2
  Sign/1 -> Compare To Constant2/1
  Compare To Constant2/1 -> Switch/2
  Abs1/1 -> Switch/1
  Logical Operator/1 -> Switch1/2
  MotCalThetae/1 -> Switch1/1
  Switch1/1 -> SinCos/1
  SinCos/1 -> Sinθ/1
  SinCos/2 -> Cosθ/1
  Switch/1 -> Switch1/3
  Add/1 -> Switch/3
  Constant1/1 -> Add/1
  Abs2/1 -> Add/2

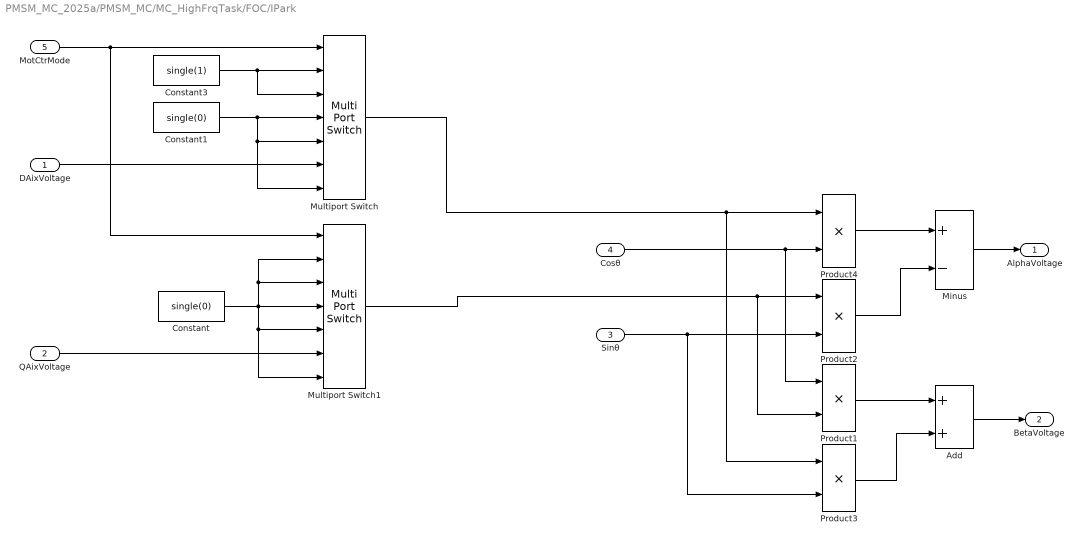
== system PMSM_MC_2025a/PMSM_MC/MC_HighFrqTask/FOC/IPark ==
  DAixVoltage : Inport
  QAixVoltage : Inport  Port=2
  Sinθ : Inport  Port=3
  Cosθ : Inport  Port=4
  MotCtrMode : Inport  Port=5
  Add : Sum
  Constant : Constant  Value=single(0)
  Constant1 : Constant  Value=single(0)
  Constant3 : Constant  Value=single(1)
  Minus : Sum  Inputs=+-
  Multiport Switch : MultiPortSwitch  Inputs=6  DiagnosticForDefault=None  SaturateOnIntegerOverflow=off  InputSameDT=off
  Multiport Switch1 : MultiPortSwitch  Inputs=6  DiagnosticForDefault=None  SaturateOnIntegerOverflow=off  InputSameDT=off
  Product{1..4} (4 alike) : Product
  AlphaVoltage : Outport
  BetaVoltage : Outport  Port=2
  wires:
  Multiport Switch/1 -> Product4/1, Product3/1
  Cosθ/1 -> Product4/2, Product1/1
  Sinθ/1 -> Product3/2, Product2/2
  Multiport Switch1/1 -> Product1/2, Product2/1
  Product4/1 -> Minus/1
  Product2/1 -> Minus/2
  Minus/1 -> AlphaVoltage/1
  Product1/1 -> Add/1
  MotCtrMode/1 -> Multiport Switch/1, Multiport Switch1/1
  QAixVoltage/1 -> Multiport Switch1/6
  DAixVoltage/1 -> Multiport Switch/6
  Product3/1 -> Add/2
  Add/1 -> BetaVoltage/1
  Constant1/1 -> Multiport Switch/7, Multiport Switch/5, Multiport Switch/4
  Constant/1 -> Multiport Switch1/2, Multiport Switch1/3, Multiport Switch1/7, Multiport Switch1/5, Multiport Switch1/4
  Constant3/1 -> Multiport Switch/3, Multiport Switch/2

== system PMSM_MC_2025a/PMSM_MC/MC_HighFrqTask/FOC/Park ==
  AlphaCurrent : Inport
  BetaCurrent : Inport  Port=2
  Sinθ : Inport  Port=3
  Cosθ : Inport  Port=4
  Add : Sum
  Add1 : Sum  Inputs=+-
  Product{,1..3} (4 alike) : Product
  DAixCurrent : Outport
  QAixCurrent : Outport  Port=2
  wires:
  Cosθ/1 -> Product2/1, Product/2
  BetaCurrent/1 -> Product1/1, Product2/2
  Sinθ/1 -> Product3/2, Product1/2
  AlphaCurrent/1 -> Product3/1, Product/1
  Product/1 -> Add/1
  Product1/1 -> Add/2
  Add/1 -> DAixCurrent/1
  Product2/1 -> Add1/1
  Product3/1 -> Add1/2
  Add1/1 -> QAixCurrent/1

== system PMSM_MC_2025a/PMSM_MC/MC_HighFrqTask/FOC/SVPWM ==
  Uα : Inport
  Uβ : Inport  Port=2
  VBus : Inport  Port=3
  SevenSegSVPWM : Subsystem
  U_H : Outport
  V_H : Outport  Port=2
  W_H : Outport  Port=3
  wires:
  Uα/1 -> SevenSegSVPWM/1(Uα)
  Uβ/1 -> SevenSegSVPWM/2(Uβ)
  VBus/1 -> SevenSegSVPWM/3(VBus)
  SevenSegSVPWM/1(UVoltage_PWM) -> U_H/1
  SevenSegSVPWM/2(VVoltage_PWM) -> V_H/1
  SevenSegSVPWM/3(WVoltage_PWM) -> W_H/1

== system PMSM_MC_2025a/PMSM_MC/MC_LowFrqTask/MotSpdCal/If Action Subsystem ==
  Ecode_cnt : Inport
  Action Port : ActionPort  ActionPortLabel=if(u1 > 8192)
  Add : Sum  Inputs=+-
  Constant : Constant  Value=int32(16384)
  EcodeCorr_cnt : Outport
  wires:
  Ecode_cnt/1 -> Add/1
  Constant/1 -> Add/2
  Add/1 -> EcodeCorr_cnt/1

== system PMSM_MC_2025a/PMSM_MC/MC_LowFrqTask/MotSpdCal/If Action Subsystem1 ==
  Ecode_cnt : Inport
  Action Port : ActionPort  ActionPortLabel=elseif(u1 < -8192)
  Add : Sum
  Constant : Constant  Value=int32(16384)
  EcodeCorr_cnt : Outport
  wires:
  Ecode_cnt/1 -> Add/1
  Constant/1 -> Add/2
  Add/1 -> EcodeCorr_cnt/1

== system PMSM_MC_2025a/PMSM_MC/MC_LowFrqTask/MotSpdCal/If Action Subsystem2 ==
  Ecode_cnt : Inport
  Action Port : ActionPort  ActionPortLabel=else
  EcodeCorr_cnt : Outport
  wires:
  Ecode_cnt/1 -> EcodeCorr_cnt/1

== system PMSM_MC_2025a/PMSM_MC/MC_LowFrqTask/MotSpdCal/LPF ==
  In : Inport
  TiCon : Inport  Port=2
  Add : Sum  Inputs=+-
  Add1 : Sum
  Constant : Constant  Value=single(1)
  Delay : Delay  DelayLength=1  InitialConditionSource=Input port
      settings: InputPortMap=u0,p4
  Product : Product
  Product1 : Product
  out : Outport
  wires:
  In/1 -> Delay/2, Product/1
  TiCon/1 -> Add/2, Product/2
  Add/1 -> Product1/1
  Constant/1 -> Add/1
  Product/1 -> Add1/1
  Product1/1 -> Add1/2
  Add1/1 -> Delay/1, out/1
  Delay/1 -> Product1/2

== system PMSM_MC_2025a/PMSM_MC/MC_HighFrqTask/ElecAngleCal/AngleCal/If Action Subsystem ==
  Ecode_PhyVal : Inport
  Action Port : ActionPort  ActionPortLabel=if(u1 == 1)
  Constant : Constant  Value=MC_POLE_NUM_CFG
  Constant1 : Constant  Value=int32(16384)
  Constant2 : Constant  Value=single(16384)
  Constant3 : Constant  Value=single(6.28)
  Data Type Conversion : DataTypeConversion  OutDataTypeStr=single  SaturateOnIntegerOverflow=off  RndMeth=Floor
  Data Type Conversion1 : DataTypeConversion  OutDataTypeStr=single  SaturateOnIntegerOverflow=off  RndMeth=Floor
  Data Type Conversion2 : DataTypeConversion  OutDataTypeStr=single  SaturateOnIntegerOverflow=off  RndMeth=Floor
  Divide : Product  Inputs=*/
  Mod : Math  Operator=mod
  Mux : Mux  Inputs=2
  Product : Product
  Product1 : Product
  Out1 : Outport
  wires:
  Ecode_PhyVal/1 -> Mod/1
  Constant1/1 -> Mod/2
  Mod/1 -> Data Type Conversion/1
  Data Type Conversion/1 -> Divide/1
  Constant2/1 -> Divide/2
  Divide/1 -> Product/1
  Constant3/1 -> Product/2
  Constant/1 -> Data Type Conversion1/1
  Data Type Conversion1/1 -> Product1/2
  Product/1 -> Product1/1, Mux/1
  Product1/1 -> Data Type Conversion2/1
  Data Type Conversion2/1 -> Mux/2
  Mux/1 -> Out1/1

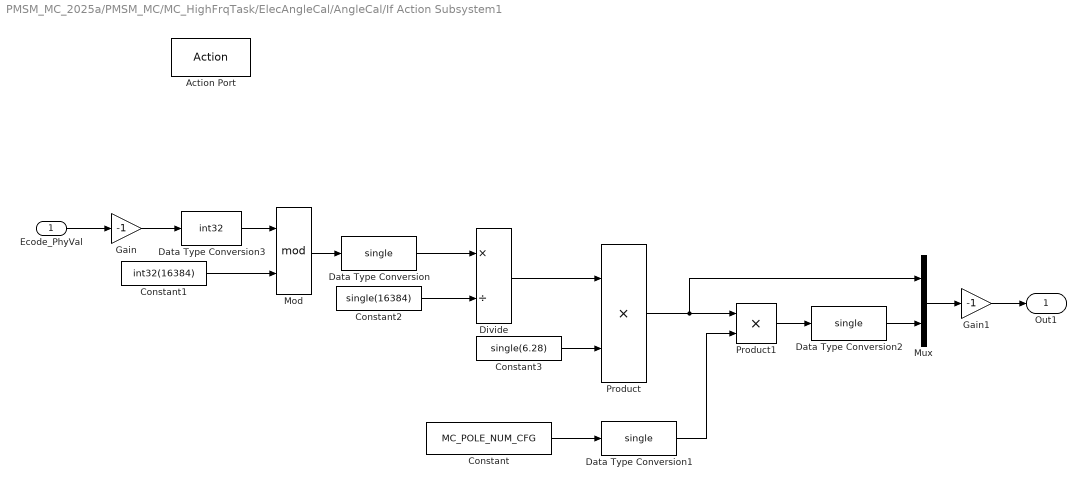
== system PMSM_MC_2025a/PMSM_MC/MC_HighFrqTask/ElecAngleCal/AngleCal/If Action Subsystem1 ==
  Ecode_PhyVal : Inport
  Action Port : ActionPort  ActionPortLabel=elseif(u1 == -1)
  Constant : Constant  Value=MC_POLE_NUM_CFG
  Constant1 : Constant  Value=int32(16384)
  Constant2 : Constant  Value=single(16384)
  Constant3 : Constant  Value=single(6.28)
  Data Type Conversion : DataTypeConversion  OutDataTypeStr=single  SaturateOnIntegerOverflow=off  RndMeth=Floor
  Data Type Conversion1 : DataTypeConversion  OutDataTypeStr=single  SaturateOnIntegerOverflow=off  RndMeth=Floor
  Data Type Conversion2 : DataTypeConversion  OutDataTypeStr=single  SaturateOnIntegerOverflow=off  RndMeth=Floor
  Data Type Conversion3 : DataTypeConversion  OutDataTypeStr=int32  SaturateOnIntegerOverflow=off  RndMeth=Floor
  Divide : Product  Inputs=*/
  Gain : Gain  Gain=-1
  Gain1 : Gain  Gain=-1
  Mod : Math  Operator=mod
  Mux : Mux  Inputs=2
  Product : Product
  Product1 : Product
  Out1 : Outport
  wires:
  Constant1/1 -> Mod/2
  Mod/1 -> Data Type Conversion/1
  Constant2/1 -> Divide/2
  Constant3/1 -> Product/2
  Data Type Conversion2/1 -> Mux/2
  Product/1 -> Product1/1, Mux/1
  Divide/1 -> Product/1
  Constant/1 -> Data Type Conversion1/1
  Data Type Conversion/1 -> Divide/1
  Product1/1 -> Data Type Conversion2/1
  Data Type Conversion1/1 -> Product1/2
  Ecode_PhyVal/1 -> Gain/1
  Gain/1 -> Data Type Conversion3/1
  Data Type Conversion3/1 -> Mod/1
  Mux/1 -> Gain1/1
  Gain1/1 -> Out1/1

== system PMSM_MC_2025a/PMSM_MC/MC_HighFrqTask/ElecAngleCal/AngleCal/If Action Subsystem2 ==
  Action Port : ActionPort  ActionPortLabel=else
  Constant : Constant  Value=single(0)
  Constant1 : Constant  Value=single(0)
  Mux : Mux  Inputs=2
  Out1 : Outport
  wires:
  Constant/1 -> Mux/1
  Constant1/1 -> Mux/2
  Mux/1 -> Out1/1

== system PMSM_MC_2025a/PMSM_MC/MC_HighFrqTask/FOC/SVPWM/SevenSegSVPWM ==
  Uα : Inport
  Uβ : Inport  Port=2
  VBus : Inport  Port=3
  Demux : Demux  Outputs=3
  SectorCaculate : Subsystem
  T1T2Caculate : Subsystem
  TcmCaculate : Subsystem
  Tpwm : Constant  Value=single(1)
  XYZCaculate : Subsystem
  UVoltage_PWM : Outport
  VVoltage_PWM : Outport  Port=2
  WVoltage_PWM : Outport  Port=3
  wires:
  Uα/1 -> SectorCaculate/1(Ualpha), XYZCaculate/1(Ualpha)
  Uβ/1 -> XYZCaculate/2(Ubeta), SectorCaculate/2(Ubeta)
  VBus/1 -> XYZCaculate/3(Udc)
  Tpwm/1 -> TcmCaculate/4(Tpwm), T1T2Caculate/3(Tpwm), XYZCaculate/4(Ts)
  SectorCaculate/1(N) -> TcmCaculate/1(N), T1T2Caculate/1(N)
  XYZCaculate/1(XYZ) -> T1T2Caculate/2(XYZ)
  T1T2Caculate/1(T1) -> TcmCaculate/2(T1)
  T1T2Caculate/2(T2) -> TcmCaculate/3(T2)
  TcmCaculate/1(Tcm1 Tcm2 Tcm3) -> Demux/1
  Demux/1 -> UVoltage_PWM/1
  Demux/2 -> VVoltage_PWM/1
  Demux/3 -> WVoltage_PWM/1

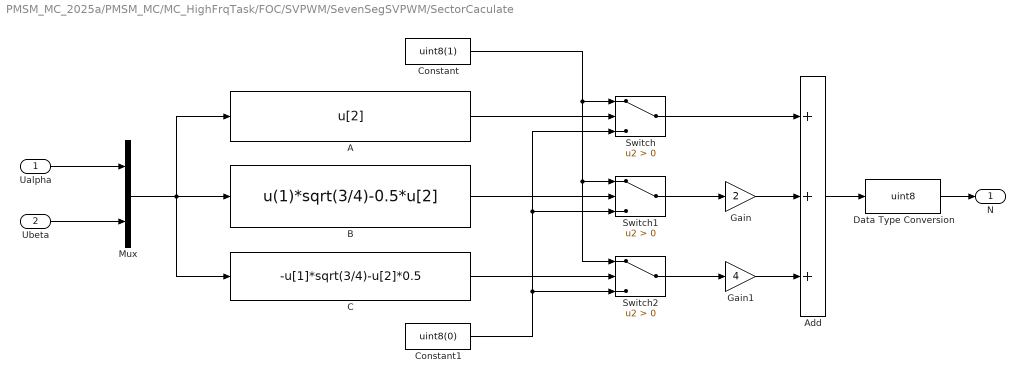
== system PMSM_MC_2025a/PMSM_MC/MC_HighFrqTask/FOC/SVPWM/SevenSegSVPWM/SectorCaculate ==
  Ualpha : Inport
  Ubeta : Inport  Port=2
  A : Fcn  Expr=u[2]
  Add : Sum  Inputs=+++
  B : Fcn  Expr=u(1)*sqrt(3/4)-0.5*u[2]
  C : Fcn  Expr=-u[1]*sqrt(3/4)-u[2]*0.5
  Constant : Constant  Value=uint8(1)
  Constant1 : Constant  Value=uint8(0)
  Data Type Conversion : DataTypeConversion  OutDataTypeStr=uint8  SaturateOnIntegerOverflow=off  RndMeth=Floor
  Gain : Gain  Gain=2
  Gain1 : Gain  Gain=4
  Mux : Mux  Inputs=2
  Switch : Switch  Criteria=u2 > Threshold  SaturateOnIntegerOverflow=off  InputSameDT=off
  Switch1 : Switch  Criteria=u2 > Threshold  SaturateOnIntegerOverflow=off  InputSameDT=off
  Switch2 : Switch  Criteria=u2 > Threshold  SaturateOnIntegerOverflow=off  InputSameDT=off
  N : Outport
  wires:
  Ualpha/1 -> Mux/1
  Ubeta/1 -> Mux/2
  Mux/1 -> C/1, A/1, B/1
  A/1 -> Switch/2
  B/1 -> Switch1/2
  C/1 -> Switch2/2
  Constant/1 -> Switch/1, Switch2/1, Switch1/1
  Constant1/1 -> Switch/3, Switch1/3, Switch2/3
  Switch2/1 -> Gain1/1
  Switch1/1 -> Gain/1
  Gain/1 -> Add/2
  Gain1/1 -> Add/3
  Switch/1 -> Add/1
  Add/1 -> Data Type Conversion/1
  Data Type Conversion/1 -> N/1

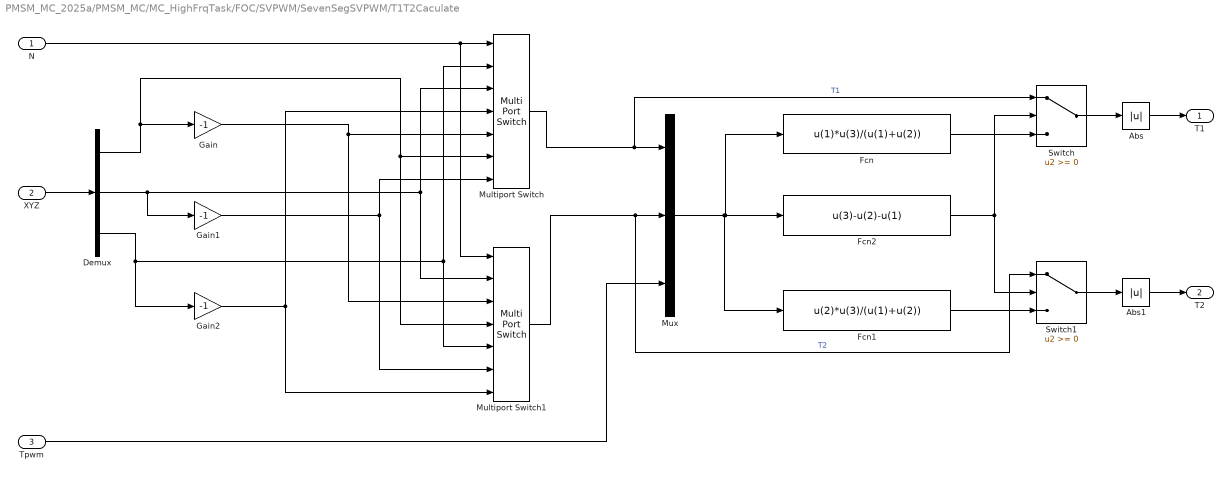
== system PMSM_MC_2025a/PMSM_MC/MC_HighFrqTask/FOC/SVPWM/SevenSegSVPWM/T1T2Caculate ==
  N : Inport
  XYZ : Inport  Port=2
  Tpwm : Inport  Port=3
  Abs : Abs  SaturateOnIntegerOverflow=off
  Abs1 : Abs  SaturateOnIntegerOverflow=off
  Demux : Demux  Outputs=3
  Fcn : Fcn  Expr=u(1)*u(3)/(u(1)+u(2))
  Fcn1 : Fcn  Expr=u(2)*u(3)/(u(1)+u(2))
  Fcn2 : Fcn  Expr=u(3)-u(2)-u(1)
  Gain : Gain  Gain=-1
  Gain1 : Gain  Gain=-1
  Gain2 : Gain  Gain=-1
  Multiport Switch : MultiPortSwitch  Inputs=6  DiagnosticForDefault=None  SaturateOnIntegerOverflow=off  InputSameDT=off
  Multiport Switch1 : MultiPortSwitch  Inputs=6  DiagnosticForDefault=None  SaturateOnIntegerOverflow=off  InputSameDT=off
  Mux : Mux  Inputs=3
  Switch : Switch  SaturateOnIntegerOverflow=off  InputSameDT=off
  Switch1 : Switch  SaturateOnIntegerOverflow=off  InputSameDT=off
  T1 : Outport
  T2 : Outport  Port=2
  wires:
  N/1 -> Multiport Switch/1, Multiport Switch1/1
  XYZ/1 -> Demux/1
  Demux/1 -> Gain/1, Multiport Switch/6, Multiport Switch1/4
  Demux/2 -> Gain1/1, Multiport Switch/3, Multiport Switch1/2
  Demux/3 -> Gain2/1, Multiport Switch1/5, Multiport Switch/2
  Gain/1 -> Multiport Switch1/3, Multiport Switch/5
  Gain2/1 -> Multiport Switch1/7, Multiport Switch/4
  Gain1/1 -> Multiport Switch/7, Multiport Switch1/6
  Multiport Switch/1 -> Switch/1, Mux/1  "T1"
  Multiport Switch1/1 -> Switch1/1, Mux/2  "T2"
  Tpwm/1 -> Mux/3
  Mux/1 -> Fcn1/1, Fcn/1, Fcn2/1
  Fcn/1 -> Switch/3
  Fcn1/1 -> Switch1/3
  Fcn2/1 -> Switch1/2, Switch/2
  Switch/1 -> Abs/1
  Abs/1 -> T1/1
  Switch1/1 -> Abs1/1
  Abs1/1 -> T2/1

== system PMSM_MC_2025a/PMSM_MC/MC_HighFrqTask/FOC/SVPWM/SevenSegSVPWM/TcmCaculate ==
  N : Inport
  T1 : Inport  Port=2
  T2 : Inport  Port=3
  Tpwm : Inport  Port=4
  Fcn : Fcn  Expr=(u(3)+u(1)+u(2))/2
  Fcn1 : Fcn  Expr=(u(3)-u(1)+u(2))/2
  Fcn2 : Fcn  Expr=(u(3)-u(1)-u(2))/2
  Multiport Switch : MultiPortSwitch  Inputs=6  DiagnosticForDefault=None  SaturateOnIntegerOverflow=off  InputSameDT=off
  Multiport Switch1 : MultiPortSwitch  Inputs=6  DiagnosticForDefault=None  SaturateOnIntegerOverflow=off  InputSameDT=off
  Multiport Switch2 : MultiPortSwitch  Inputs=6  DiagnosticForDefault=None  SaturateOnIntegerOverflow=off  InputSameDT=off
  Mux : Mux  Inputs=3
  Mux1 : Mux  Inputs=3
  Tcm1 Tcm2 Tcm3 : Outport
  wires:
  Mux/1 -> Tcm1 Tcm2 Tcm3/1
  T2/1 -> Mux1/2
  T1/1 -> Mux1/1
  Tpwm/1 -> Mux1/3
  Mux1/1 -> Fcn/1, Fcn2/1, Fcn1/1
  N/1 -> Multiport Switch2/1, Multiport Switch1/1, Multiport Switch/1
  Fcn1/1 -> Multiport Switch1/4, Multiport Switch/7, Multiport Switch/2, Multiport Switch1/5, Multiport Switch2/6, Multiport Switch2/3
  Fcn/1 -> Multiport Switch1/6, Multiport Switch2/7, Multiport Switch2/5, Multiport Switch/4, Multiport Switch/3, Multiport Switch1/2
  Fcn2/1 -> Multiport Switch1/7, Multiport Switch/6, Multiport Switch/5, Multiport Switch1/3, Multiport Switch2/4, Multiport Switch2/2
  Multiport Switch/1 -> Mux/1
  Multiport Switch1/1 -> Mux/2
  Multiport Switch2/1 -> Mux/3

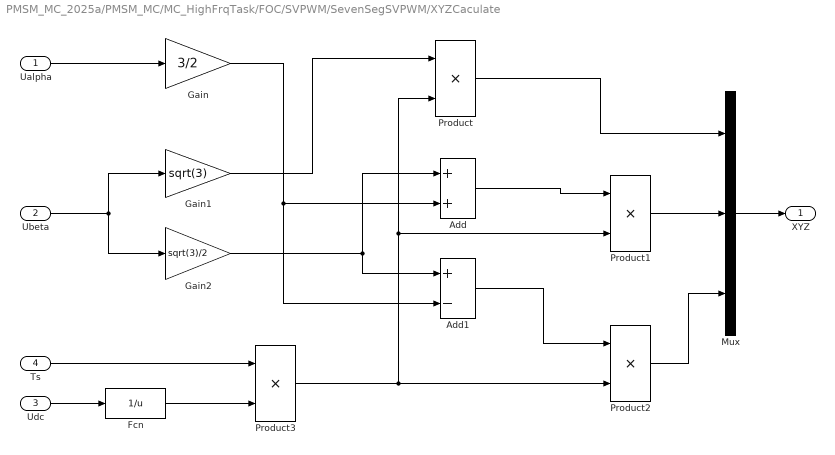
== system PMSM_MC_2025a/PMSM_MC/MC_HighFrqTask/FOC/SVPWM/SevenSegSVPWM/XYZCaculate ==
  Ualpha : Inport
  Ubeta : Inport  Port=2
  Udc : Inport  Port=3
  Ts : Inport  Port=4
  Add : Sum
  Add1 : Sum  Inputs=+-
  Fcn : Fcn  Expr=1/u
  Gain : Gain  Gain=3/2
  Gain1 : Gain  Gain=sqrt(3)
  Gain2 : Gain  Gain=sqrt(3)/2
  Mux : Mux  Inputs=3
  Product{,1..3} (4 alike) : Product
  XYZ : Outport
  wires:
  Ualpha/1 -> Gain/1
  Ubeta/1 -> Gain2/1, Gain1/1
  Gain/1 -> Add/2, Add1/2
  Gain1/1 -> Product/1
  Gain2/1 -> Add1/1, Add/1
  Ts/1 -> Product3/1
  Product3/1 -> Product1/2, Product/2, Product2/2
  Add/1 -> Product1/1
  Udc/1 -> Fcn/1
  Fcn/1 -> Product3/2
  Add1/1 -> Product2/1
  Product1/1 -> Mux/2
  Product2/1 -> Mux/3
  Product/1 -> Mux/1
  Mux/1 -> XYZ/1

== stateflow chart PMSM_MC_2025a/PMSM_MC/MC_LowFrqTask/MotModeCtr/Chart ==
  state Calibrate
    state Init
      en:
      MotCtrMode=0;
    state Calibrate1
      en:
      MotCtrMode=1;
      MotCalThetae = 0;//0°
    state Calibrate2
      en:
      MotOffsetBuff[0]=Ecode_cnt;
      MotCtrMode=2;
      MotCalThetae = 0;//0°
    state RngChk
      en:
      MotOffsetBuff[1]=Ecode_cnt;
      RangeCheck();
    (default) -> Init
    Init -> Calibrate1 : [MotorSpdRef != 0]
    Calibrate1 -> Calibrate2 : [after(1.5,sec)]
    Calibrate2 -> RngChk : [after(1.5,sec)]
  state RangeCheck [function]
    (default) -> (junction 21)
    (junction 21) -> (junction 23) [order 1] : [abs(MotOffsetBuff[0]-MotOffsetBuff[1])>100]
    (junction 21) -> (junction 24) [order 2] : {
        | MotCalNormal=1;
        | MotOffset = (MotOffsetBuff[0]+MotOffsetBuff[1])/2;
        | }
    (junction 23) -> (junction 25) : {MotCalNormal=0;}
    (junction 25) -> (junction 24)
    (junction 24) -> (junction 35)
  state CalFailed
    en:
    MotCtrMode=3;
  state Normal
    state Stop
      en:
      MotCtrMode=4;
    state Run
      en:
      MotCtrMode=5;
    (default) -> Stop
    Run -> Stop : [MotorSpdRef==0]
    Stop -> Run : [MotorSpdRef!=0]
  (default) -> Calibrate
  CalFailed -> Calibrate : [MotorSpdRef==0]
  RngChk -> CalFailed [order 1] : [MotCalNormal==0]
  RngChk -> Normal [order 2] : [MotCalNormal==1]
  data: MotCtrMode output uint8; Ecode_cnt input int32; MotorSpdRef input int16; MotOffset output int32; MotCalThetae output single; MotOffsetBuff local int32 size=2; MotCalNormal local boolean

== stateflow chart PMSM_MC_2025a/Scheduler ==
  (default) -> (junction 6)
  (junction 6) -> (junction 11) [order 1] : [counter%%20==19]
  (junction 6) -> (junction 10) [order 2]
  (junction 11) -> (junction 9) : {trig_MidFrq_1ms;}
  (junction 9) -> (junction 10)
  (junction 10) -> (junction 18) : {trig_HighFrq_50us;}
  (junction 18) -> (junction 20) [order 1] : [counter>=100000000]
  (junction 18) -> (junction 24) [order 2] : {counter++;}
  (junction 20) -> (junction 22) : {counter=0;}
  (junction 22) -> (junction 24)
  (junction 24) -> (junction 27)
  data: counter local uint32 =0
  events: trig_MidFrq_1ms output FUNCTION_CALL_EVENT; trig_HighFrq_50us output FUNCTION_CALL_EVENT
